simulink model "Q2 – Linear Convolution"  (R2024b)
settings: Solver=VariableStepAuto  StartTime=0.0  StopTime=10.0  RelTol=1e-3
libraries: dspsigops x1
settings Model: Creator=sobha  LastModifiedBy=sobha

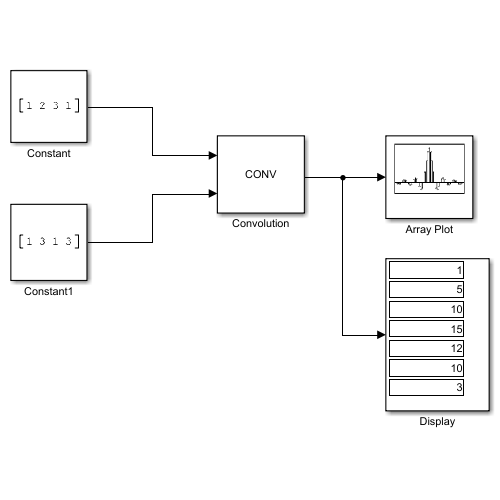
[thumbnail: Simulink's stored preview of the top-level diagram]
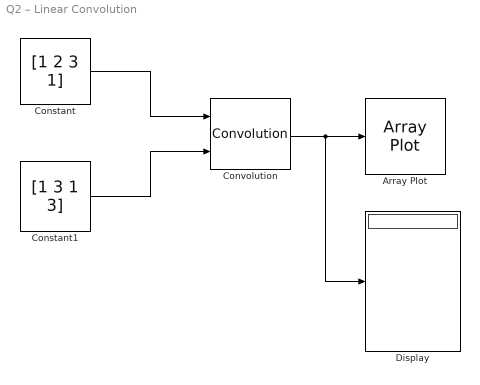
== system Q2 – Linear Convolution ==
  Array Plot : ArrayPlot  WindowPosition=[764.000000,374.000000,398.000000,376.000000,]  ScopeFrameLocation=window  YLimits=[-0.75 16.75]
  Constant : Constant  Value=[1 2 3 1]  SampleTime=1
  Constant1 : Constant  Value=[1 3 1 3]  SampleTime=1
  Convolution : dspsigops/Convolution  domain=Time  roundingMode=Floor  overflowMode=off  outputDataTypeStr=Inherit: Same as accumulator  outputMin=[]  outputMax=[]  outputLastDataTypeStr=Inherit: Same as accumulator
  Display : Display
  wires:
  Constant/1 -> Convolution/1
  Constant1/1 -> Convolution/2
  Convolution/1 -> Display/1, Array Plot/1
